simulink model "HW5"  (R2022b)
settings: Solver=VariableStepAuto  StartTime=0.0  StopTime=1000  FixedStep=0.0001  RelTol=1e-3
libraries: simulink x5
settings Model: Creator=ali14  LastModifiedBy=ali14

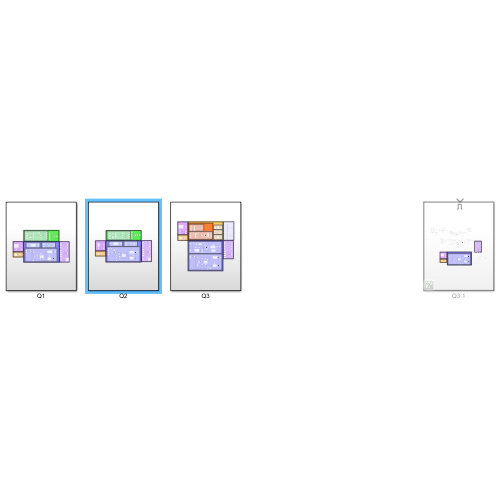
[thumbnail: Simulink's stored preview of the top-level diagram]
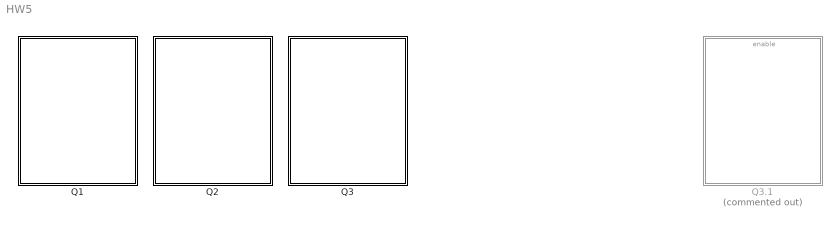
== system HW5 ==
  Q1 : Subsystem
  Q2 : Subsystem
  Q3 : Subsystem
  Q3.1 : Subsystem  Commented=on

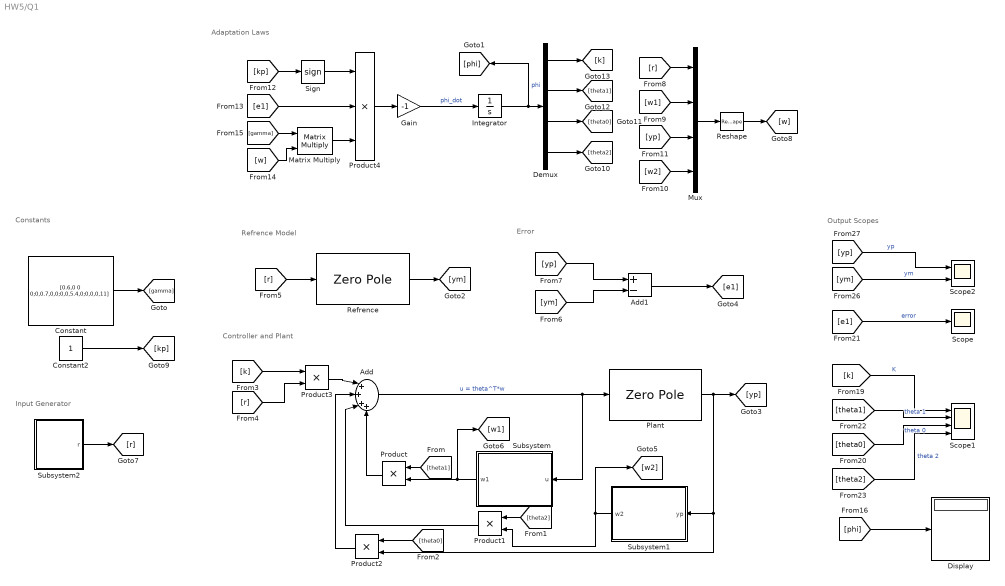
== system HW5/Q1 ==
  note: Constants
  note: Input Generator
  note: Adaptation Laws
  note: Controller and Plant
  note: Error
  note: Refrence Model
  note: Output Scopes
  Add : Sum  Inputs=|++++
  Add1 : Sum  Inputs=+-
  Constant : Constant  Value=[0.6,0 0 0;0,0.7,0,0;0,0,5.4,0;0,0,0,11]
  Constant2 : Constant
  Demux : Demux
  Display : Display
  Gain : Gain  Gain=-1
  Integrator : Integrator
  Matrix Multiply : Product  Multiplication=Matrix(*)
  Mux : Mux
  Plant : ZeroPole  Zeros=[-1]  Poles=[2 1]  Gain=1
  Product{,1..3} (4 alike) : Product
  Product4 : Product  Inputs=3
  Refrence : ZeroPole  Zeros=[]  Poles=[-1]  Gain=1
  Reshape : Reshape  OutputDimensionality=Column vector (2-D)
  Scope : Scope
  Scope1 : Scope  NumInputPorts=4
  Scope2 : Scope  NumInputPorts=2
  Sign : Signum
  Subsystem : Subsystem
  Subsystem1 : Subsystem
  Subsystem2 : Subsystem
  wires:
  Demux/1 -> [k]
  Subsystem1/1(w2) -> Product1/2, [w2]
  [theta2] -> Product1/1
  Demux/4 -> [theta2]
  Plant/1 -> [yp], Product2/2, Subsystem1/1(yp)
  Constant2/1 -> [kp]
  Refrence/1 -> [ym]
  [kp] -> Sign/1
  [r] -> Refrence/1
  [w1] -> Mux/2
  Reshape/1 -> [w]
  Sign/1 -> Product4/1
  [k] -> Product3/1
  Add1/1 -> [e1]
  Product1/1 -> Add/3
  [yp] -> Add1/1
  Product2/1 -> Add/2
  [theta1] -> Product/1
  Subsystem/1(w1) -> [w1], Product/2
  Add/1 -> Subsystem/1(u), Plant/1  "u = theta^T*w"
  Product/1 -> Add/4
  Mux/1 -> Reshape/1
  [w2] -> Mux/4
  Demux/3 -> [theta0]
  [r] -> Product3/2
  Product3/1 -> Add/1
  [ym] -> Add1/2
  [theta0] -> Product2/1
  Gain/1 -> Integrator/1  "phi_dot"
  Product4/1 -> Gain/1
  [r] -> Mux/1
  Integrator/1 -> [phi], Demux/1  "phi"
  Demux/2 -> [theta1]
  Subsystem2/1(r) -> [r]
  [e1] -> Product4/2
  [yp] -> Mux/3
  Constant/1 -> [gamma]
  [w] -> Matrix Multiply/2
  Matrix Multiply/1 -> Product4/3
  [gamma] -> Matrix Multiply/1
  [yp] -> Scope2/1  "yp"
  [theta1] -> Scope1/2  "theta 1"
  [theta0] -> Scope1/3  "theta 0"
  [theta2] -> Scope1/4  "theta 2"
  [e1] -> Scope/1  "error"
  [ym] -> Scope2/2  "ym"
  [k] -> Scope1/1  "K"
  [phi] -> Display/1

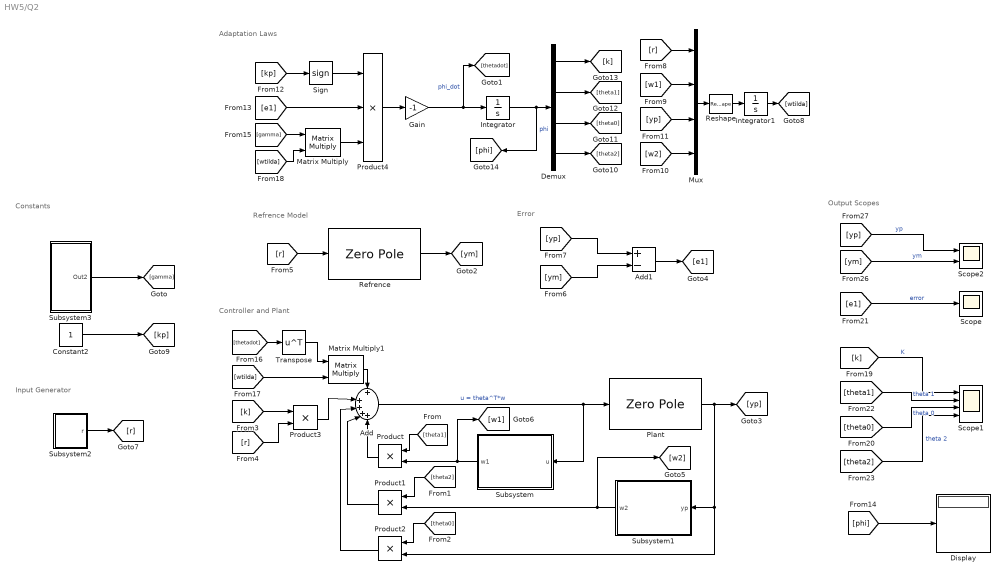
== system HW5/Q2 ==
  note: Constants
  note: Input Generator
  note: Adaptation Laws
  note: Controller and Plant
  note: Error
  note: Refrence Model
  note: Output Scopes
  Add : Sum  Inputs=+|++++
  Add1 : Sum  Inputs=+-
  Constant2 : Constant
  Demux : Demux
  Display : Display
  Gain : Gain  Gain=-1
  Integrator : Integrator
  Integrator1 : Integrator
  Matrix Multiply : Product  Multiplication=Matrix(*)
  Matrix Multiply1 : Product  Multiplication=Matrix(*)
  Mux : Mux
  Plant : ZeroPole  Zeros=[]  Gain=1
  Product{,1..3} (4 alike) : Product
  Product4 : Product  Inputs=3
  Refrence : ZeroPole  Zeros=[]  Poles=[-1 -1]  Gain=1
  Reshape : Reshape  OutputDimensionality=Column vector (2-D)
  Scope : Scope
  Scope1 : Scope  NumInputPorts=4
  Scope2 : Scope  NumInputPorts=2
  Sign : Signum
  Subsystem : Subsystem
  Subsystem1 : Subsystem
  Subsystem2 : Subsystem
  Subsystem3 : Subsystem
  Transpose : Math  Operator=transpose
  wires:
  Demux/1 -> [k]
  Subsystem1/1(w2) -> Product1/2, [w2]
  [theta2] -> Product1/1
  Demux/4 -> [theta2]
  Plant/1 -> [yp], Product2/2, Subsystem1/1(yp)
  Constant2/1 -> [kp]
  Refrence/1 -> [ym]
  [kp] -> Sign/1
  [r] -> Refrence/1
  [w1] -> Mux/2
  Sign/1 -> Product4/1
  [k] -> Product3/1
  Add1/1 -> [e1]
  [yp] -> Add1/1
  [theta1] -> Product/1
  Subsystem/1(w1) -> [w1], Product/2
  Add/1 -> Subsystem/1(u), Plant/1  "u = theta^T*w"
  Mux/1 -> Reshape/1
  [w2] -> Mux/4
  Demux/3 -> [theta0]
  [r] -> Product3/2
  [ym] -> Add1/2
  [theta0] -> Product2/1
  Gain/1 -> [thetadot], Integrator/1  "phi_dot"
  Product4/1 -> Gain/1
  [r] -> Mux/1
  Integrator/1 -> [phi], Demux/1  "phi"
  Demux/2 -> [theta1]
  Subsystem2/1(r) -> [r]
  [e1] -> Product4/2
  [yp] -> Mux/3
  [wtilda] -> Matrix Multiply/2
  Matrix Multiply/1 -> Product4/3
  [gamma] -> Matrix Multiply/1
  [yp] -> Scope2/1  "yp"
  [theta1] -> Scope1/2  "theta 1"
  [theta0] -> Scope1/3  "theta 0"
  [theta2] -> Scope1/4  "theta 2"
  [e1] -> Scope/1  "error"
  [ym] -> Scope2/2  "ym"
  [k] -> Scope1/1  "K"
  Reshape/1 -> Integrator1/1
  Integrator1/1 -> [wtilda]
  Transpose/1 -> Matrix Multiply1/1
  [wtilda] -> Matrix Multiply1/2
  [thetadot] -> Transpose/1
  Product/1 -> Add/5
  Product1/1 -> Add/4
  Product2/1 -> Add/3
  Product3/1 -> Add/2
  Matrix Multiply1/1 -> Add/1
  [phi] -> Display/1
  Subsystem3/1(Out2) -> [gamma]

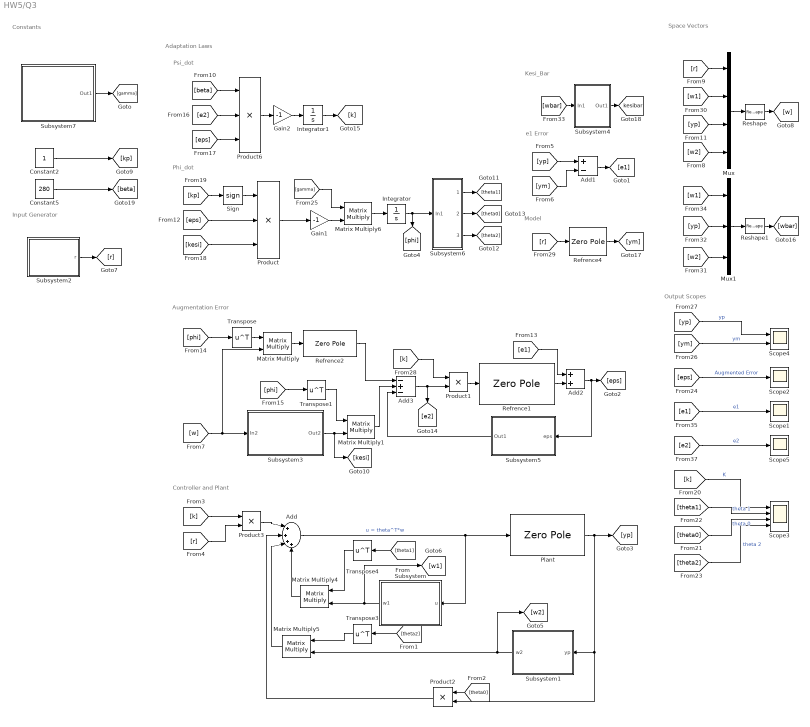
== system HW5/Q3 ==
  note: Space Vectors
  note: Kesi_Bar
  note: e1 Error
  note: Model
  note: Augmentation Error
  note: Phi_dot
  note: Psi_dot
  note: Adaptation Laws
  note: Controller and Plant
  note: Input Generator
  note: Constants
  note: Output Scopes
  Add : Sum  Inputs=|++++
  Add1 : Sum  Inputs=+-
  Add2 : Sum
  Add3 : Sum  Inputs=-+-
  Constant2 : Constant
  Constant5 : Constant  Value=280
  Gain1 : Gain  Gain=-1
  Gain2 : Gain  Gain=-1
  Integrator : Integrator
  Integrator1 : Integrator  InitialCondition=0.2
  Matrix Multiply{,1,4..6} (5 alike) : Product  Multiplication=Matrix(*)
  Mux : Mux
  Mux1 : Mux  Inputs=3
  Plant : ZeroPole  Zeros=[]  Poles=[-1 -2 -3]  Gain=1
  Product : Product  Inputs=3
  Product1 : Product
  Product2 : Product
  Product3 : Product
  Product6 : Product  Inputs=3
  Refrence1 : ZeroPole  Zeros=[]  Poles=[ -4]  Gain=64
  Refrence2 : ZeroPole  Zeros=[]  Poles=[ -4 -4]  Gain=1
  Refrence4 : ZeroPole  Zeros=[]  Poles=[-4 -4 -4]  Gain=64
  Reshape : Reshape  OutputDimensionality=Column vector (2-D)
  Reshape1 : Reshape  OutputDimensionality=Column vector (2-D)
  Scope1 : Scope
  Scope2 : Scope
  Scope3 : Scope  NumInputPorts=4
  Scope4 : Scope  NumInputPorts=2
  Scope5 : Scope
  Sign : Signum
  Subsystem : Subsystem
  Subsystem1 : Subsystem
  Subsystem2 : Subsystem
  Subsystem3 : Subsystem
  Subsystem4 : Subsystem
  Subsystem5 : Subsystem
  Subsystem6 : Subsystem
  Subsystem7 : Subsystem
  Transpose{,1,3..4} (4 alike) : Math  Operator=transpose
  tag scope: kesibar=global
  wires:
  Matrix Multiply5/1 -> Add/3
  Subsystem1/1(w2) -> [w2], Matrix Multiply5/2
  Transpose3/1 -> Matrix Multiply5/1
  [theta2] -> Transpose3/1
  [theta1] -> Transpose4/1
  Product3/1 -> Add/1
  Add/1 -> Subsystem/1(u), Plant/1  "u = theta^T*w"
  Transpose4/1 -> Matrix Multiply4/1
  [theta0] -> Product2/1
  [k] -> Product3/1
  [r] -> Product3/2
  Subsystem/1(w1) -> [w1], Matrix Multiply4/2
  Matrix Multiply4/1 -> Add/4
  Plant/1 -> [yp], Product2/2, Subsystem1/1(yp)
  Product2/1 -> Add/2
  Subsystem2/1(r) -> [r]
  Constant2/1 -> [kp]
  Refrence4/1 -> [ym]
  [r] -> Refrence4/1
  [yp] -> Add1/1
  [ym] -> Add1/2
  Add1/1 -> [e1]
  [w] -> Subsystem3/1(In2), Matrix Multiply/2
  Add2/1 -> Subsystem5/1(eps), [eps]
  [e1] -> Add2/1
  Matrix Multiply/1 -> Refrence2/1
  [phi] -> Transpose/1
  Transpose/1 -> Matrix Multiply/1
  [phi] -> Transpose1/1
  Transpose1/1 -> Matrix Multiply1/1
  Refrence2/1 -> Add3/1
  Matrix Multiply1/1 -> Add3/2
  Add3/1 -> Product1/2, [e2]
  [kesi] -> Product/3
  Product/1 -> Gain1/1
  Integrator/1 -> Subsystem6/1(In1), [phi]
  Gain2/1 -> Integrator1/1
  Product6/1 -> Gain2/1
  [eps] -> Product/2
  [kp] -> Sign/1
  Sign/1 -> Product/1
  [theta0] -> Scope3/3  "theta 0"
  [eps] -> Scope2/1  "Augmented Error"
  [theta2] -> Scope3/4  "theta 2"
  [theta1] -> Scope3/2  "theta 1"
  [yp] -> Scope4/1  "yp"
  [k] -> Scope3/1  "K"
  [ym] -> Scope4/2  "ym"
  Matrix Multiply6/1 -> Integrator/1
  Gain1/1 -> Matrix Multiply6/2
  [gamma] -> Matrix Multiply6/1
  [eps] -> Product6/3
  [e2] -> Product6/2
  [beta] -> Product6/1
  Refrence1/1 -> Add2/2
  Product1/1 -> Refrence1/1
  [k] -> Product1/1
  [yp] -> Mux/3
  [r] -> Mux/1
  [w1] -> Mux/2
  Mux/1 -> Reshape/1
  Reshape/1 -> [w]
  [w2] -> Mux/4
  Mux1/1 -> Reshape1/1
  Reshape1/1 -> [wbar]
  [w2] -> Mux1/3
  [yp] -> Mux1/2
  [w1] -> Mux1/1
  [wbar] -> Subsystem4/1(In1)
  Subsystem4/1(Out1) -> [kesibar]
  Subsystem5/1(Out1) -> Add3/3
  Subsystem3/1(Out2) -> [kesi], Matrix Multiply1/2
  Constant5/1 -> [beta]
  [e1] -> Scope1/1  "e1"
  Integrator1/1 -> [k]
  Subsystem6/1(Out1) -> [theta1]
  Subsystem6/2(Out2) -> [theta0]
  Subsystem6/3(Out3) -> [theta2]
  Subsystem7/1(Out1) -> [gamma]
  [e2] -> Scope5/1  "e2"

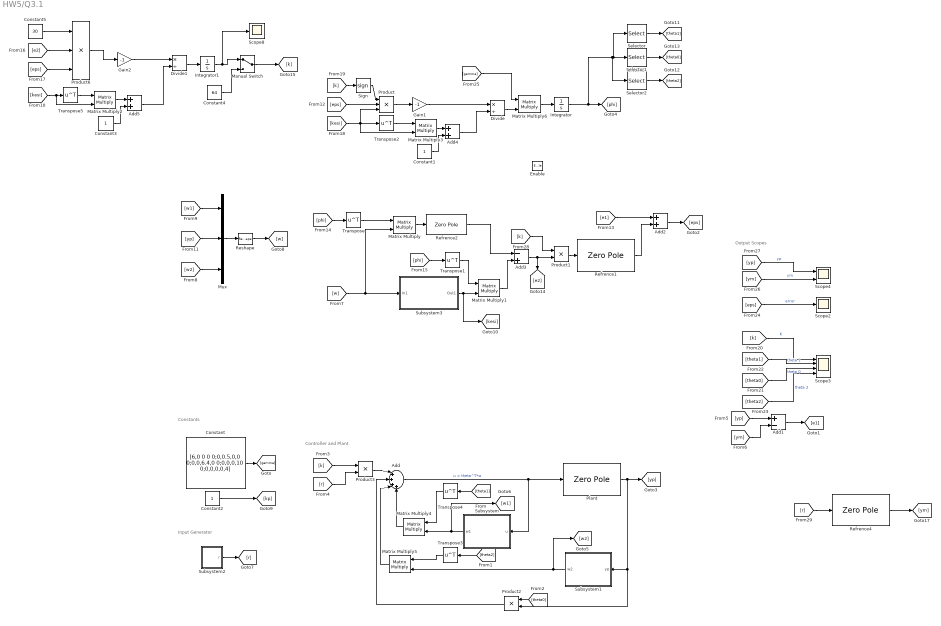
== system HW5/Q3.1 ==
  note: Controller and Plant
  note: Input Generator
  note: Constants
  note: Output Scopes
  Enable : EnablePort
  Add : Sum  Inputs=|++++
  Add1 : Sum  Inputs=+-
  Add2 : Sum
  Add3 : Sum  Inputs=-+
  Add4 : Sum
  Add5 : Sum
  Constant : Constant  Value=[6,0 0 0 0;0,0.5,0,0 0;0,0,6.4,0 0;0,0,0,10 0;0,0,0,0,4]
  Constant1 : Constant
  Constant2 : Constant
  Constant3 : Constant
  Constant4 : Constant  Value=64
  Constant5 : Constant  Value=30
  Divide : Product  Inputs=*/
  Divide1 : Product  Inputs=*/
  Gain1 : Gain  Gain=-1
  Gain2 : Gain  Gain=-1
  Integrator : Integrator
  Integrator1 : Integrator  InitialCondition=2
  Manual Switch : ManualSwitch
  Matrix Multiply{,1..6} (7 alike) : Product  Multiplication=Matrix(*)
  Mux : Mux  Inputs=3
  Plant : ZeroPole  Zeros=[]  Poles=[-1 -2 -3]  Gain=1
  Product : Product  Inputs=3
  Product1 : Product
  Product2 : Product
  Product3 : Product
  Product6 : Product  Inputs=3
  Refrence1 : ZeroPole  Zeros=[]  Poles=[ -4]  Gain=64
  Refrence2 : ZeroPole  Zeros=[]  Poles=[ -4 -4]  Gain=1
  Refrence4 : ZeroPole  Zeros=[]  Poles=[-4 -4 -4]  Gain=64
  Reshape : Reshape  OutputDimensionality=Column vector (2-D)
  Scope2 : Scope
  Scope3 : Scope  NumInputPorts=4
  Scope4 : Scope  NumInputPorts=2
  Scope8 : Scope
  Selector : Selector  InputPortWidth=5  IndexOptions=Index vector (dialog)  Indices=[1 2]  OutputSizes=1
  Selector1 : Selector  InputPortWidth=5  IndexOptions=Index vector (dialog)  Indices=[3]  OutputSizes=1
  Selector2 : Selector  InputPortWidth=5  IndexOptions=Index vector (dialog)  Indices=[4 5]  OutputSizes=1
  Sign : Signum
  Subsystem : Subsystem
  Subsystem1 : Subsystem
  Subsystem2 : Subsystem
  Subsystem3 : Subsystem
  Transpose{,1..5} (6 alike) : Math  Operator=transpose
  wires:
  Matrix Multiply5/1 -> Add/3
  Subsystem1/1(w2) -> [w2], Matrix Multiply5/2
  Transpose3/1 -> Matrix Multiply5/1
  [theta2] -> Transpose3/1
  [theta1] -> Transpose4/1
  Product3/1 -> Add/1
  Add/1 -> Subsystem/1(u), Plant/1  "u = theta^T*w"
  Transpose4/1 -> Matrix Multiply4/1
  [theta0] -> Product2/1
  [k] -> Product3/1
  [r] -> Product3/2
  Subsystem/1(w1) -> [w1], Matrix Multiply4/2
  Matrix Multiply4/1 -> Add/4
  Plant/1 -> [yp], Product2/2, Subsystem1/1(yp)
  Product2/1 -> Add/2
  Subsystem2/1(r) -> [r]
  Constant/1 -> [gamma]
  Constant2/1 -> [kp]
  Refrence4/1 -> [ym]
  [r] -> Refrence4/1
  [yp] -> Add1/1
  [ym] -> Add1/2
  Add1/1 -> [e1]
  [w2] -> Mux/3
  [yp] -> Mux/2
  Mux/1 -> Reshape/1
  Reshape/1 -> [w]
  [w] -> Matrix Multiply/2, Subsystem3/1(In1)
  Add2/1 -> [eps]
  [e1] -> Add2/1
  Matrix Multiply/1 -> Refrence2/1
  [phi] -> Transpose/1
  Transpose/1 -> Matrix Multiply/1
  [phi] -> Transpose1/1
  Transpose1/1 -> Matrix Multiply1/1
  Subsystem3/1(Out1) -> [kesi], Matrix Multiply1/2
  Refrence2/1 -> Add3/1
  Matrix Multiply1/1 -> Add3/2
  Add3/1 -> Product1/2, [e2]
  [w1] -> Mux/1
  [kesi] -> Matrix Multiply3/2, Transpose2/1, Product/3
  Product/1 -> Gain1/1
  Gain1/1 -> Divide/1
  Transpose2/1 -> Matrix Multiply3/1
  Matrix Multiply3/1 -> Add4/1
  Constant1/1 -> Add4/2
  Add4/1 -> Divide/2
  Integrator/1 -> [phi], Selector2/1, Selector/1, Selector1/1
  Integrator1/1 -> Scope8/1, Manual Switch/1
  Divide1/1 -> Integrator1/1
  Constant4/1 -> Manual Switch/2
  Gain2/1 -> Divide1/1
  Manual Switch/1 -> [k]
  Product6/1 -> Gain2/1
  [eps] -> Product/2
  [k] -> Sign/1
  Sign/1 -> Product/1
  Constant3/1 -> Add5/2
  Matrix Multiply2/1 -> Add5/1
  [kesi] -> Matrix Multiply2/2, Transpose5/1
  Add5/1 -> Divide1/2
  Transpose5/1 -> Matrix Multiply2/1
  [theta0] -> Scope3/3  "theta 0"
  [eps] -> Scope2/1  "error"
  [theta2] -> Scope3/4  "theta 2"
  [theta1] -> Scope3/2  "theta 1"
  [yp] -> Scope4/1  "yp"
  [k] -> Scope3/1  "K"
  [ym] -> Scope4/2  "ym"
  Selector/1 -> [theta1]
  Selector1/1 -> [theta0]
  Selector2/1 -> [theta2]
  Matrix Multiply6/1 -> Integrator/1
  Divide/1 -> Matrix Multiply6/2
  [gamma] -> Matrix Multiply6/1
  [eps] -> Product6/3
  [e2] -> Product6/2
  Constant5/1 -> Product6/1
  Refrence1/1 -> Add2/2
  Product1/1 -> Refrence1/1
  [k] -> Product1/1

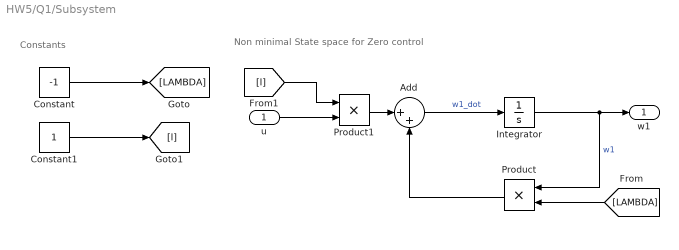
== system HW5/Q1/Subsystem ==
  note: Non minimal State space for Zero control
  note: Constants
  u : Inport
  Add : Sum  Inputs=|++
  Constant : Constant  Value=-1
  Constant1 : Constant
  Integrator : Integrator
  Product : Product
  Product1 : Product
  w1 : Outport
  wires:
  Integrator/1 -> Product/1, w1/1  "w1"
  Add/1 -> Integrator/1  "w1_dot"
  [LAMBDA] -> Product/2
  Product/1 -> Add/2
  [l] -> Product1/1
  Product1/1 -> Add/1
  u/1 -> Product1/2
  Constant1/1 -> [l]
  Constant/1 -> [LAMBDA]

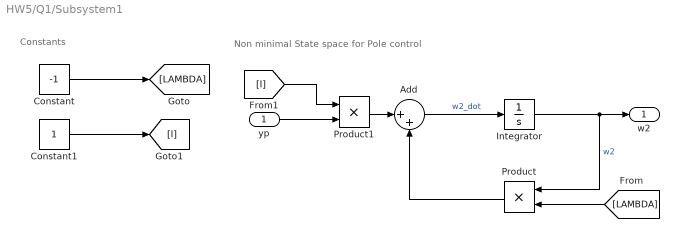
== system HW5/Q1/Subsystem1 ==
  note: Constants
  note: Non minimal State space for Pole control
  yp : Inport
  Add : Sum  Inputs=|++
  Constant : Constant  Value=-1
  Constant1 : Constant
  Integrator : Integrator
  Product : Product
  Product1 : Product
  w2 : Outport
  wires:
  Constant1/1 -> [l]
  Constant/1 -> [LAMBDA]
  [LAMBDA] -> Product/2
  [l] -> Product1/1
  Product1/1 -> Add/1
  Integrator/1 -> Product/1, w2/1  "w2"
  yp/1 -> Product1/2
  Add/1 -> Integrator/1  "w2_dot"
  Product/1 -> Add/2

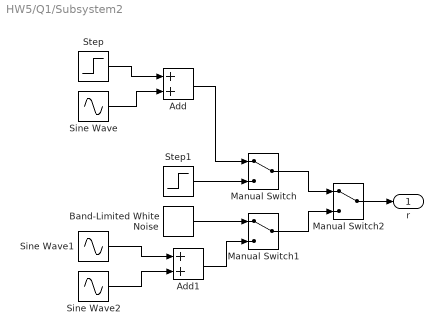
== system HW5/Q1/Subsystem2 ==
  Add : Sum
  Add1 : Sum
  Band-Limited White Noise : simulink/Sources/Band-Limited White Noise  Cov=[0.1]  Ts=0.1  seed=[23341]
  Manual Switch : ManualSwitch
  Manual Switch1 : ManualSwitch
  Manual Switch2 : ManualSwitch
  Sine Wave : Sin  SampleTime=0
  Sine Wave1 : Sin  SampleTime=0
  Sine Wave2 : Sin  Frequency=4  SampleTime=0
  Step : Step  Time=0  SampleTime=0
  Step1 : Step  SampleTime=0
  r : Outport
  wires:
  Add/1 -> Manual Switch/1
  Step/1 -> Add/1
  Sine Wave/1 -> Add/2
  Step1/1 -> Manual Switch/2
  Manual Switch2/1 -> r/1
  Manual Switch/1 -> Manual Switch2/1
  Manual Switch1/1 -> Manual Switch2/2
  Band-Limited White Noise/1 -> Manual Switch1/1
  Add1/1 -> Manual Switch1/2
  Sine Wave1/1 -> Add1/1
  Sine Wave2/1 -> Add1/2

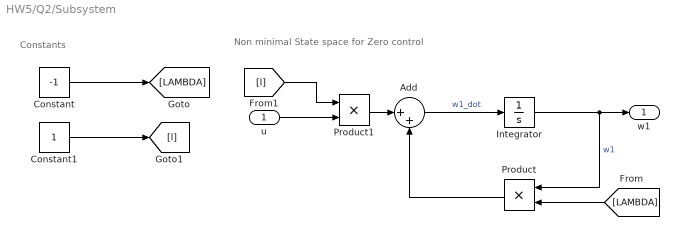
== system HW5/Q2/Subsystem ==
  note: Non minimal State space for Zero control
  note: Constants
  u : Inport
  Add : Sum  Inputs=|++
  Constant : Constant  Value=-1
  Constant1 : Constant
  Integrator : Integrator
  Product : Product
  Product1 : Product
  w1 : Outport
  wires:
  Integrator/1 -> Product/1, w1/1  "w1"
  Add/1 -> Integrator/1  "w1_dot"
  [LAMBDA] -> Product/2
  Product/1 -> Add/2
  [l] -> Product1/1
  Product1/1 -> Add/1
  u/1 -> Product1/2
  Constant1/1 -> [l]
  Constant/1 -> [LAMBDA]

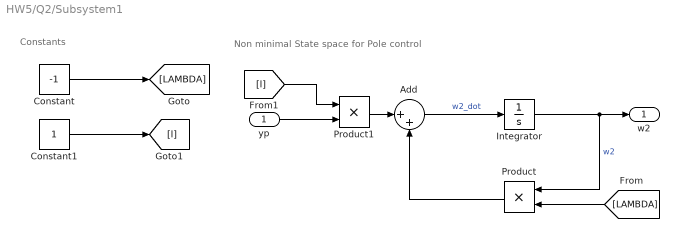
== system HW5/Q2/Subsystem1 ==
  note: Constants
  note: Non minimal State space for Pole control
  yp : Inport
  Add : Sum  Inputs=|++
  Constant : Constant  Value=-1
  Constant1 : Constant
  Integrator : Integrator
  Product : Product
  Product1 : Product
  w2 : Outport
  wires:
  Constant1/1 -> [l]
  Constant/1 -> [LAMBDA]
  [LAMBDA] -> Product/2
  [l] -> Product1/1
  Product1/1 -> Add/1
  Integrator/1 -> Product/1, w2/1  "w2"
  yp/1 -> Product1/2
  Add/1 -> Integrator/1  "w2_dot"
  Product/1 -> Add/2

== system HW5/Q2/Subsystem2 ==
  Add : Sum
  Band-Limited White Noise : simulink/Sources/Band-Limited White Noise  Cov=[0.1]  Ts=0.1  seed=[23341]
  Manual Switch : ManualSwitch  CurrentSetting=0
  Manual Switch1 : ManualSwitch
  Manual Switch2 : ManualSwitch
  Sine Wave : Sin  SampleTime=0
  Step : Step  Time=0  SampleTime=0
  Step1 : Step  SampleTime=0
  r : Outport
  wires:
  Add/1 -> Manual Switch/1
  Step/1 -> Add/1
  Sine Wave/1 -> Add/2
  Step1/1 -> Manual Switch/2
  Manual Switch2/1 -> r/1
  Manual Switch/1 -> Manual Switch2/1
  Manual Switch1/1 -> Manual Switch2/2
  Band-Limited White Noise/1 -> Manual Switch1/1

== system HW5/Q2/Subsystem3 ==
  Manual Switch : ManualSwitch
  Parameter : Constant  Value=[43,0 0 0;0,34,0,0;0,0,45,0;0,0,0,13]
  Sine : Constant  Value=[4,0 0 0;0,95,0,0;0,0,20,0;0,0,0,7]
  Out2 : Outport
  wires:
  Parameter/1 -> Manual Switch/2
  Manual Switch/1 -> Out2/1
  Sine/1 -> Manual Switch/1

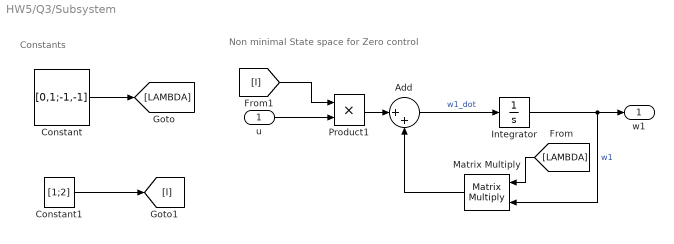
== system HW5/Q3/Subsystem ==
  note: Non minimal State space for Zero control
  note: Constants
  u : Inport
  Add : Sum  Inputs=|++
  Constant : Constant  Value=[0,1;-1,-1]
  Constant1 : Constant  Value=[1;2]  VectorParams1D=off
  Integrator : Integrator
  Matrix Multiply : Product  Multiplication=Matrix(*)
  Product1 : Product
  w1 : Outport
  wires:
  Integrator/1 -> Matrix Multiply/2, w1/1  "w1"
  Add/1 -> Integrator/1  "w1_dot"
  Matrix Multiply/1 -> Add/2
  [l] -> Product1/1
  Product1/1 -> Add/1
  u/1 -> Product1/2
  Constant1/1 -> [l]
  Constant/1 -> [LAMBDA]
  [LAMBDA] -> Matrix Multiply/1

== system HW5/Q3/Subsystem1 ==
  note: Non minimal State space for Pole control
  note: Constants
  yp : Inport
  Add : Sum  Inputs=|++
  Constant : Constant  Value=[0,1;-1,-1]
  Constant1 : Constant  Value=[1;2]  VectorParams1D=off
  Integrator : Integrator
  Matrix Multiply : Product  Multiplication=Matrix(*)
  Product1 : Product
  w2 : Outport
  wires:
  [l] -> Product1/1
  Product1/1 -> Add/1
  Integrator/1 -> Matrix Multiply/2, w2/1  "w2"
  yp/1 -> Product1/2
  Add/1 -> Integrator/1  "w2_dot"
  Constant/1 -> [LAMBDA]
  Constant1/1 -> [l]
  [LAMBDA] -> Matrix Multiply/1
  Matrix Multiply/1 -> Add/2

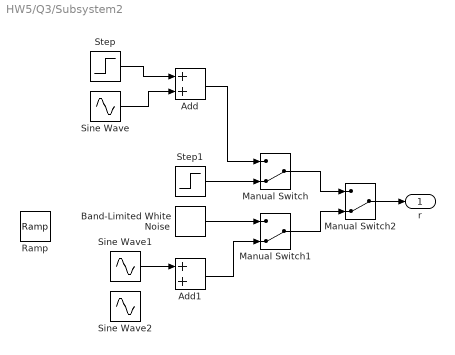
== system HW5/Q3/Subsystem2 ==
  Add : Sum
  Add1 : Sum
  Band-Limited White Noise : simulink/Sources/Band-Limited White Noise  Cov=[0.1]  Ts=0.1  seed=[23341]
  Manual Switch : ManualSwitch  CurrentSetting=0
  Manual Switch1 : ManualSwitch  CurrentSetting=0
  Manual Switch2 : ManualSwitch  CurrentSetting=0
  Ramp : simulink/Sources/Ramp  slope=1  start=0  InitialOutput=0
  Sine Wave : Sin  Amplitude=6  SampleTime=0
  Sine Wave1 : Sin  SampleTime=0
  Sine Wave2 : Sin  Frequency=0.5  SampleTime=0
  Step : Step  Time=0  SampleTime=0
  Step1 : Step  SampleTime=0
  r : Outport
  wires:
  Add/1 -> Manual Switch/1
  Step/1 -> Add/1
  Sine Wave/1 -> Add/2
  Step1/1 -> Manual Switch/2
  Manual Switch2/1 -> r/1
  Manual Switch/1 -> Manual Switch2/1
  Manual Switch1/1 -> Manual Switch2/2
  Band-Limited White Noise/1 -> Manual Switch1/1
  Add1/1 -> Manual Switch1/2
  Sine Wave1/1 -> Add1/1

== system HW5/Q3/Subsystem3 ==
  In2 : Inport
  Demux1 : Demux  Outputs=6
  Mux1 : Mux  Inputs=6
  Refrence{1,6..10} (6 alike) : ZeroPole  Zeros=[]  Poles=[ -4 -4]  Gain=1
  Reshape1 : Reshape  OutputDimensionality=Column vector (2-D)
  Out2 : Outport
  wires:
  Mux1/1 -> Reshape1/1
  ? -> ?
  Refrence8/1 -> Mux1/4
  Demux1/3 -> Refrence7/1
  Reshape1/1 -> Out2/1
  ? -> ?
  Demux1/2 -> Refrence6/1
  In2/1 -> Demux1/1
  Demux1/4 -> Refrence8/1
  Demux1/5 -> Refrence10/1
  Refrence10/1 -> Mux1/5
  Refrence7/1 -> Mux1/3
  Refrence9/1 -> Mux1/1
  Refrence6/1 -> Mux1/2
  Demux1/1 -> Refrence9/1
  Demux1/6 -> Refrence1/1
  Refrence1/1 -> Mux1/6

== system HW5/Q3/Subsystem4 ==
  In1 : Inport
  Demux : Demux  Outputs=5
  Mux : Mux  Inputs=5
  Refrence{1..5} (5 alike) : ZeroPole  Zeros=[]  Poles=[ -4 -4]  Gain=1
  Reshape : Reshape  OutputDimensionality=Column vector (2-D)
  Out1 : Outport
  wires:
  Demux/1 -> Refrence4/1
  Demux/2 -> Refrence1/1
  Demux/3 -> Refrence2/1
  Demux/4 -> Refrence3/1
  Refrence3/1 -> Mux/4
  Refrence2/1 -> Mux/3
  Refrence1/1 -> Mux/2
  Refrence4/1 -> Mux/1
  In1/1 -> Demux/1
  Demux/5 -> Refrence5/1
  Refrence5/1 -> Mux/5
  Mux/1 -> Reshape/1
  Reshape/1 -> Out1/1

== system HW5/Q3/Subsystem5 ==
  eps : Inport
  Matrix Multiply : Product  Multiplication=Matrix(*)
  Product : Product
  Transpose : Math  Operator=transpose
  Out1 : Outport
  wires:
  [kesibar] -> Matrix Multiply/2, Transpose/1
  Transpose/1 -> Matrix Multiply/1
  Matrix Multiply/1 -> Product/1
  Product/1 -> Out1/1
  eps/1 -> Product/2

== system HW5/Q3/Subsystem6 ==
  In1 : Inport
  Selector : Selector  InputPortWidth=6  IndexOptions=Index vector (dialog)  Indices=[2 3]  OutputSizes=1
  Selector1 : Selector  InputPortWidth=6  IndexOptions=Index vector (dialog)  Indices=[4]  OutputSizes=1
  Selector2 : Selector  InputPortWidth=6  IndexOptions=Index vector (dialog)  Indices=[5 6]  OutputSizes=1
  Out1 : Outport
  Out2 : Outport  Port=2
  Out3 : Outport  Port=3
  wires:
  Selector1/1 -> Out2/1
  In1/1 -> Selector1/1, Selector/1, Selector2/1
  Selector/1 -> Out1/1
  Selector2/1 -> Out3/1

== system HW5/Q3/Subsystem7 ==
  Constant : Constant  Value=[3,0 0 0 0 0;0,4,0,0 0 0;0,0,5,0 0 0;0,0,0,4 0 0;0,0,0,0,30 0;0,0,0,0,0 60]
  Constant1 : Constant  Value=[10,0 0 0 0 0;0,40,0,0 0 0;0,0,50,0 0 0;0,0,0,70 0 0;0,0,0,0,10 0;0,0,0,0,0 10]
  Manual Switch : ManualSwitch
  Out1 : Outport
  wires:
  Constant/1 -> Manual Switch/1
  Constant1/1 -> Manual Switch/2
  Manual Switch/1 -> Out1/1

== system HW5/Q3.1/Subsystem ==
  note: Non minimal State space for Zero control
  note: Constants
  u : Inport
  Add : Sum  Inputs=|++
  Constant : Constant  Value=[0,1;-1,-1]
  Constant1 : Constant  Value=[1;2]  VectorParams1D=off
  Integrator : Integrator
  Matrix Multiply : Product  Multiplication=Matrix(*)
  Product1 : Product
  w1 : Outport
  wires:
  Integrator/1 -> Matrix Multiply/2, w1/1  "w1"
  Add/1 -> Integrator/1  "w1_dot"
  Matrix Multiply/1 -> Add/2
  [l] -> Product1/1
  Product1/1 -> Add/1
  u/1 -> Product1/2
  Constant1/1 -> [l]
  Constant/1 -> [LAMBDA]
  [LAMBDA] -> Matrix Multiply/1

== system HW5/Q3.1/Subsystem1 ==
  note: Non minimal State space for Pole control
  note: Constants
  yp : Inport
  Add : Sum  Inputs=|++
  Constant : Constant  Value=[0,1;-1,-1]
  Constant1 : Constant  Value=[1;2]  VectorParams1D=off
  Integrator : Integrator
  Matrix Multiply : Product  Multiplication=Matrix(*)
  Product1 : Product
  w2 : Outport
  wires:
  [l] -> Product1/1
  Product1/1 -> Add/1
  Integrator/1 -> Matrix Multiply/2, w2/1  "w2"
  yp/1 -> Product1/2
  Add/1 -> Integrator/1  "w2_dot"
  Constant/1 -> [LAMBDA]
  Constant1/1 -> [l]
  [LAMBDA] -> Matrix Multiply/1
  Matrix Multiply/1 -> Add/2

== system HW5/Q3.1/Subsystem2 ==
  Add : Sum
  Band-Limited White Noise : simulink/Sources/Band-Limited White Noise  Cov=[0.1]  Ts=0.1  seed=[23341]
  Manual Switch : ManualSwitch
  Manual Switch1 : ManualSwitch
  Manual Switch2 : ManualSwitch  CurrentSetting=0
  Sine Wave : Sin  Amplitude=6  SampleTime=0
  Step : Step  Time=0  SampleTime=0
  Step1 : Step  Time=0  SampleTime=0
  r : Outport
  wires:
  Add/1 -> Manual Switch/1
  Step/1 -> Add/1
  Sine Wave/1 -> Add/2
  Step1/1 -> Manual Switch/2
  Manual Switch2/1 -> r/1
  Manual Switch/1 -> Manual Switch2/1
  Manual Switch1/1 -> Manual Switch2/2
  Band-Limited White Noise/1 -> Manual Switch1/1

== system HW5/Q3.1/Subsystem3 ==
  In1 : Inport
  Demux : Demux  Outputs=5
  Mux : Mux  Inputs=5
  Refrence{1..5} (5 alike) : ZeroPole  Zeros=[]  Poles=[ -4 -4]  Gain=1
  Reshape : Reshape  OutputDimensionality=Column vector (2-D)
  Out1 : Outport
  wires:
  Demux/1 -> Refrence4/1
  Demux/2 -> Refrence1/1
  Demux/3 -> Refrence2/1
  Demux/4 -> Refrence3/1
  Refrence3/1 -> Mux/4
  Refrence2/1 -> Mux/3
  Refrence1/1 -> Mux/2
  Refrence4/1 -> Mux/1
  In1/1 -> Demux/1
  Demux/5 -> Refrence5/1
  Refrence5/1 -> Mux/5
  Mux/1 -> Reshape/1
  Reshape/1 -> Out1/1
